simulink model "solar_mppt_hdl_ready"  (R2026a)
settings: Solver=FixedStepAuto  StopTime=1.0  FixedStep=1e-5
values from neighbouring files (symbols this model uses):
  irradiance_day = pchip(t_coarse, irradiance_coarse, t_sim)    [flc_init.m]
  t_sim = linspace(0, 1.0, 1001)    [flc_init.m]
undefined symbols (not defined in the file or in its folder): DiscIntNeverNeededParam
libraries: nesl_utility x5, fl_lib x4, ee_lib x2, sl_discontinuities x1
settings Model: Creator=user  LastModifiedBy=user
settings OptimizationCC: ConditionallyExecuteInputs=off
settings DebuggingCC: AlgebraicLoopMsg=error
settings HardwareCC: ProdHWDeviceType=ASIC/FPGA->ASIC/FPGA  TargetBitPerPointer=64.0  TargetBitPerSizeT=64.0  TargetBitPerPtrDiffT=64.0  TargetLongLongMode=on  TargetIntDivRoundTo=Zero  TargetEndianess=LittleEndian  TargetWordSize=64.0  TargetHWDeviceType=Custom Processor->MATLAB Host Computer  ProdEqTarget=off

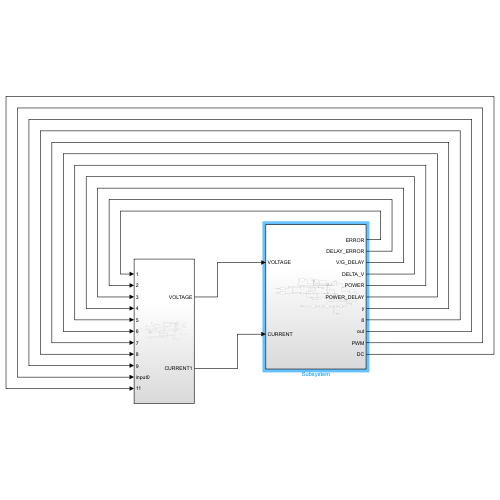
[thumbnail: Simulink's stored preview of the top-level diagram]
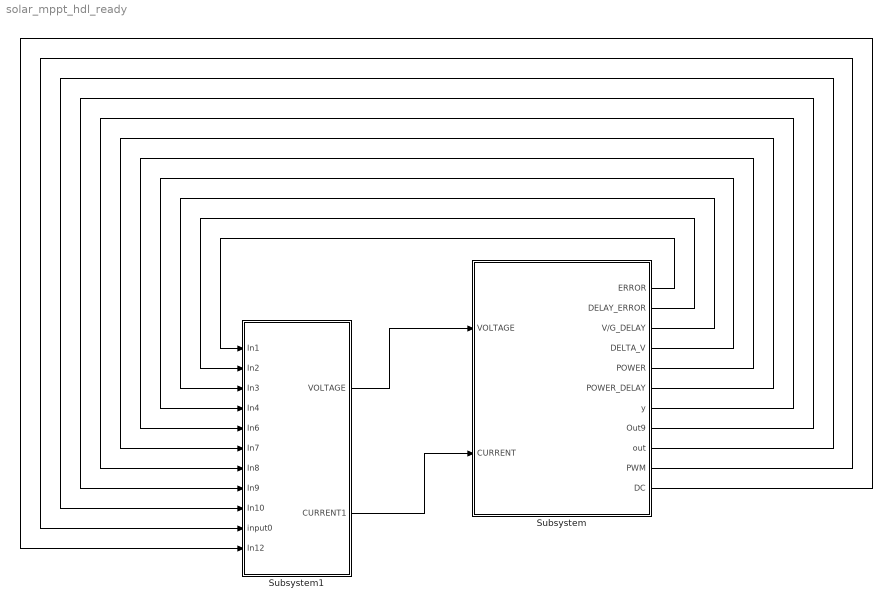
== system solar_mppt_hdl_ready ==
  Subsystem : Subsystem
  Subsystem1 : Subsystem
  wires:
  Subsystem/1(ERROR) -> Subsystem1/1(In1)
  Subsystem/2(DELAY_ERROR) -> Subsystem1/2(In2)
  Subsystem/3(V/G_DELAY) -> Subsystem1/3(In3)
  Subsystem/4(DELTA_V) -> Subsystem1/4(In4)
  Subsystem/5(POWER) -> Subsystem1/5(In6)
  Subsystem/6(POWER_DELAY) -> Subsystem1/6(In7)
  Subsystem/7(y) -> Subsystem1/7(In8)
  Subsystem/8(Out9) -> Subsystem1/8(In9)
  Subsystem/9(out) -> Subsystem1/9(In10)
  Subsystem/10(PWM) -> Subsystem1/10(input0)
  Subsystem/11(DC) -> Subsystem1/11(In12)
  Subsystem1/1(VOLTAGE) -> Subsystem/1(VOLTAGE)
  Subsystem1/2(CURRENT1) -> Subsystem/2(CURRENT)

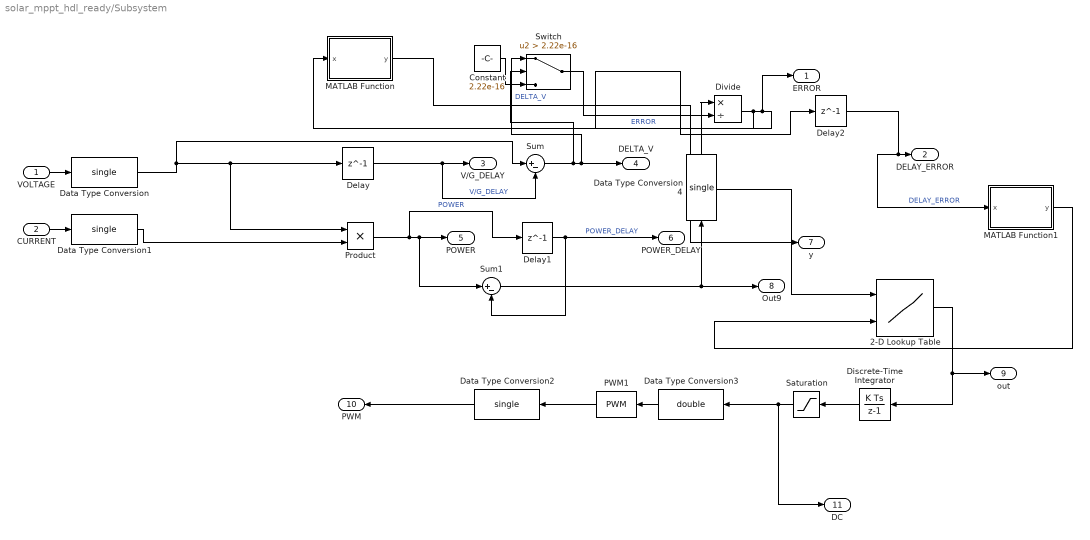
== system solar_mppt_hdl_ready/Subsystem ==
  VOLTAGE : Inport  SampleTime=1e-5
  CURRENT : Inport  Port=2  SampleTime=1e-5
  2-D Lookup Table : Lookup_n-D  BreakpointsForDimension1=[1:3]  BreakpointsForDimension2=[1:3]  InternalRulePriority=Speed  OutDataTypeStr=single  RndMeth=Simplest
      settings: InputPortMap=u0,u1
  Constant : Constant  Value=2.22e-16  OutDataTypeStr=single
  Data Type Conversion{,1..2,4} (4 alike) : DataTypeConversion  OutDataTypeStr=single  SaturateOnIntegerOverflow=off  RndMeth=Floor
  Data Type Conversion3 : DataTypeConversion  OutDataTypeStr=double  SaturateOnIntegerOverflow=off  RndMeth=Floor
  Delay : Delay  DelayLength=1  InitialCondition=0  InputProcessing=Columns as channels (frame based)
  Delay1 : Delay  DelayLength=1  InitialCondition=0  InputProcessing=Columns as channels (frame based)
  Delay2 : Delay  DelayLength=1  InitialCondition=0  InputProcessing=Columns as channels (frame based)
  Discrete-Time Integrator : DiscreteIntegrator  InitialCondition=0.4  SampleTime=-1  ICPrevOutput=DiscIntNeverNeededParam  ICPrevScaledInput=DiscIntNeverNeededParam
  Divide : Product  Inputs=*/
  MATLAB Function : MATLAB Function  TreatAsAtomicUnit=on
  MATLAB Function1 : MATLAB Function  TreatAsAtomicUnit=on
  PWM1 : sl_discontinuities/PWM  DisableCoverage=on  Period=1  InitialDelay=0  DisallowZeroDutyCycle=off  RunAtFixedTimeIntervals=on  SampleTime=1e-5
      settings: LibrarySourceBlock=simulink/Discontinuities/PWM
  Product : Product
  Saturation : Saturate  UpperLimit=0.9  LowerLimit=0.05  OutDataTypeStr=single
  Sum : Sum  Inputs=|+-
  Sum1 : Sum  Inputs=|+-
  Switch : Switch  Criteria=u2 > Threshold  Threshold=2.22e-16  SaturateOnIntegerOverflow=off  InputSameDT=off
  ERROR : Outport
  DELAY_ERROR : Outport  Port=2
  V/G_DELAY : Outport  Port=3
  DELTA_V : Outport  Port=4
  POWER : Outport  Port=5
  POWER_DELAY : Outport  Port=6
  y : Outport  Port=7
  Out9 : Outport  Port=8
  out : Outport  Port=9
  PWM : Outport  Port=10
  DC : Outport  Port=11
  wires:
  MATLAB Function/1(y) -> 2-D Lookup Table/1, y/1
  Discrete-Time Integrator/1 -> Saturation/1
  Saturation/1 -> Data Type Conversion3/1, DC/1
  MATLAB Function1/1(y) -> 2-D Lookup Table/2
  Sum/1 -> Switch/2, DELTA_V/1, Switch/1  "DELTA_V"
  Switch/1 -> Divide/2
  Delay1/1 -> POWER_DELAY/1, Sum1/2  "POWER_DELAY"
  Product/1 -> Delay1/1, POWER/1, Sum1/1  "POWER"
  Divide/1 -> MATLAB Function/1(x), ERROR/1, Delay2/1  "ERROR"
  Constant/1 -> Switch/3
  Sum1/1 -> Out9/1, Data Type Conversion4/1
  Delay/1 -> V/G_DELAY/1, Sum/2  "V/G_DELAY"
  PWM1/1 -> Data Type Conversion2/1
  2-D Lookup Table/1 -> out/1, Discrete-Time Integrator/1
  CURRENT/1 -> Data Type Conversion1/1
  Delay2/1 -> MATLAB Function1/1(x), DELAY_ERROR/1  "DELAY_ERROR"
  VOLTAGE/1 -> Data Type Conversion/1
  Data Type Conversion/1 -> Product/1, Delay/1, Sum/1
  Data Type Conversion1/1 -> Product/2
  Data Type Conversion3/1 -> PWM1/1
  Data Type Conversion2/1 -> PWM/1
  Data Type Conversion4/1 -> Divide/1

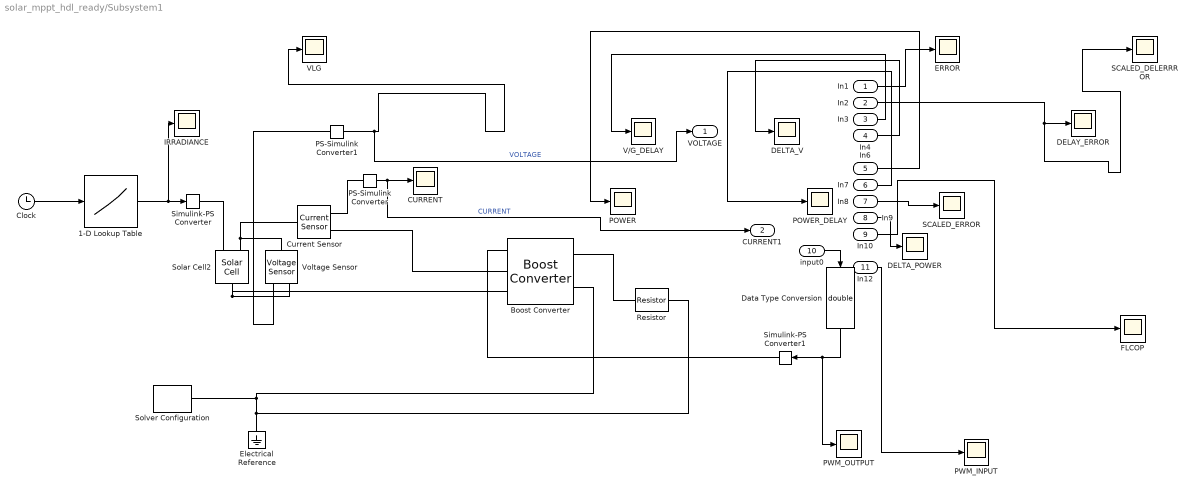
== system solar_mppt_hdl_ready/Subsystem1 ==
  In1 : Inport
  In2 : Inport  Port=2
  In3 : Inport  Port=3
  In4 : Inport  Port=4
  In6 : Inport  Port=5
  In7 : Inport  Port=6
  In8 : Inport  Port=7
  In9 : Inport  Port=8
  In10 : Inport  Port=9
  input0 : Inport  Port=10
  In12 : Inport  Port=11
  1-D Lookup Table : Lookup_n-D  NumberOfTableDimensions=1  BreakpointsForDimension1=t_sim  Table=irradiance_day  ExtrapMethod=Clip  InternalRulePriority=Speed  RndMeth=Simplest
  Boost Converter : ee_lib/Semiconductors & Converters/Converters/Boost Converter  port_option=ee.enum.controlport.ps  device_type=ee.enum.converters.switchingdevice.ideal  Vf=0.8 V  Ron=0.001 Ohm  Rds=0.001 Ohm  Goff=1e-5 1/Ohm  Vgt=1 V  Vgt_off=-1 V  Ih=1 A  Vth=6 V  K=0  diode_param=ee.enum.converters.protectiondiode.nodynamics  diode_Vf=0.8 V  diode_Ron=0.001 Ohm  diode_Goff=1e-5 1/Ohm  diode_C=50 nF  diode_iRM=-235 A  diode_iF=300 A  diode_idot=-50 A/us  diode_trr_param=ee.enum.converters.diodetrr.trr_factor  diode_trr_factor=3  diode_trr=15 us  diode_Qrr=1500 s*uA  Lf=1e-6 H  Rl=0 Ohm  Cf=1e-7 F  Rf=1e-6 Ohm  snubber_type=ee.enum.converters.snubber.exclude  Cs=1e-7 F  Rs=0.1 Ohm  iL_specify=off  iL_priority=High  iL=0 A  iL_nominal_specify=off  iL_nominal_value=1  iL_nominal_unit=A  vc_specify=off  vc_priority=High  vc=0 V  vc_nominal_specify=off  vc_nominal_value=1  vc_nominal_unit=V
  CURRENT : Scope
      settings: ActiveDisplayYMinimum=-0.41351020650465781  ActiveDisplayYMaximum=3.7215920776010369
  Clock : Clock
  Current Sensor : fl_lib/Electrical/Electrical Sensors/Current Sensor
  DELAY_ERROR : Scope
      settings: ActiveDisplayYMinimum=-0.932438052271241  ActiveDisplayYMaximum=7.5437756032088767  DataLoggingVariableName=ScopeData8
  DELTA_POWER : Scope
      settings: DataLoggingVariableName=ScopeData6
  DELTA_V : Scope
      settings: ActiveDisplayYMinimum=-1  ActiveDisplayYMaximum=1  DataLoggingVariableName=ScopeData3
  Data Type Conversion : DataTypeConversion  OutDataTypeStr=double  SaturateOnIntegerOverflow=off  RndMeth=Floor
  ERROR : Scope
      settings: ActiveDisplayYMinimum=-0.932438052271241  ActiveDisplayYMaximum=7.5437756032088767  DataLoggingVariableName=ScopeData7
  Electrical Reference : fl_lib/Electrical/Electrical Elements/Electrical Reference
  FLCOP : Scope
      settings: ActiveDisplayYMinimum=-1  ActiveDisplayYMaximum=1  DataLoggingVariableName=ScopeData9
  IRRADIANCE : Scope
      settings: ActiveDisplayYMinimum=-124.88690159999997  ActiveDisplayYMaximum=1124.9821144  DataLoggingVariableName=ScopeData16
  POWER : Scope
      settings: ActiveDisplayYMinimum=-1  ActiveDisplayYMaximum=1  DataLoggingVariableName=ScopeData4
  POWER_DELAY : Scope
      settings: Title=Output Power  ActiveDisplayYMinimum=-14.008631000583797  ActiveDisplayYMaximum=126.07767900525421  YLabel=Power Po(in watts)  DataLoggingVariableName=Po  DataLoggingSaveFormat=Array
  PS-Simulink Converter : nesl_utility/PS-Simulink Converter  PhysicalDomain=network_engine_domain  SubClassName=ps_output  LeftPortType=input  RightPortType=output  PseudoPeriodic=off  Frequencies=[]  VectorFormat=inherit  Unit=inherit  AffineConversion=off
  PS-Simulink Converter1 : nesl_utility/PS-Simulink Converter  PhysicalDomain=network_engine_domain  SubClassName=ps_output  LeftPortType=input  RightPortType=output  PseudoPeriodic=off  Frequencies=[]  VectorFormat=inherit  Unit=inherit  AffineConversion=off
  PWM_INPUT : Scope
      settings: ActiveDisplayYMinimum=-1  ActiveDisplayYMaximum=1  DataLoggingVariableName=ScopeData12
  PWM_OUTPUT : Scope
      settings: ActiveDisplayYMinimum=-1  ActiveDisplayYMaximum=1  DataLoggingVariableName=ScopeData11
  Resistor : fl_lib/Electrical/Electrical Elements/Resistor  R=10 Ohm  i_specify=off  i_priority=None  i=0 A  i_nominal_specify=off  i_nominal_value=1  i_nominal_unit=A  v_specify=off  v_priority=None  v=0 V  v_nominal_specify=off  v_nominal_value=1  v_nominal_unit=V
  SCALED_DELERRROR : Scope
      settings: ActiveDisplayYMinimum=-1  ActiveDisplayYMaximum=1  DataLoggingVariableName=ScopeData14
  SCALED_ERROR : Scope
      settings: ActiveDisplayYMinimum=-1  ActiveDisplayYMaximum=1  DataLoggingVariableName=ScopeData13
  Simulink-PS Converter : nesl_utility/Simulink-PS Converter  PhysicalDomain=network_engine_domain  SubClassName=ps_input  LeftPortType=input  RightPortType=output  PseudoPeriodic=off  Frequencies=[]  NoiseDistribution=none  NoiseParameters=[]  Unit=1  AffineConversion=off  FilteringAndDerivatives=provide  SimscapeFilterOrder=1  InputFilterTimeConstant=0.001  UdotUserProvided=0
  Simulink-PS Converter1 : nesl_utility/Simulink-PS Converter  PhysicalDomain=network_engine_domain  SubClassName=ps_input  LeftPortType=input  RightPortType=output  PseudoPeriodic=off  Frequencies=[]  NoiseDistribution=none  NoiseParameters=[]  Unit=1  AffineConversion=off  FilteringAndDerivatives=provide  SimscapeFilterOrder=1  InputFilterTimeConstant=0.001  UdotUserProvided=0
  Solar Cell2 : ee_lib/Sources/Solar Cell  prm=ee.enum.sources.solar_cell_prm.eightParameter  Isc=7.34 A  Voc=21.5 V  Is=1e-10 A  Is2=1e-10 A  Iph=7.34 A  Ir0=1000 W/m^2  ec=1.5  N2=2  Rs=0 Ohm  Rp=inf Ohm  N_series=36  N_parallel=1  TIPH1=0 1/K  EG=1.11 eV  TXIS1=3  TXIS2=3  TRS1=0  TRP1=0  Tmeas=25 degC  TFIXED=25 degC  thermal_mass=100 J/K  initial_temperature=25 degC
  Solver Configuration : nesl_utility/Solver Configuration  PhysicalDomain=network_engine_domain  SubClassName=solver  LeftPortType=input  RightPortType=generic  Tones=[]  Harmonics=[]  SimulateNoise=off  Profile=off  UseLocalSampling=off  EnableSwitchedLinearOptims=on  FrequencyDomain=off  UseCCode=off  RelTol=0.001  AbsTol=0.001  MinStep=1e-09  ToWorkspace=off  RevertToSquareIcSolve=off  NumHomotopyIterations=100  PhasorMode=off  PhasorModeNumHarmonics=1  ConsistencySolver=NEWTON_XTOL_AFTER_FTOL  CanonicalOrdering=CANONICAL  OptimizeIntermediates=OPTIMIZED  IndexReductionMethod=DerivativeReplacement  DoDC=off  ResidualTolerance=1e-09  ConsistencyTolSource=GLOBAL  ConsistencyAbsTol=0.001  ConsistencyRelTol=0.001  ConsistencyTolFactor=0.001  UseLocalSolver=off  LocalSolverChoice=NE_BACKWARD_EULER_ADVANCER  ResolveIndetEquations=on  FunctionEvalNumThread=1  LocalSolverSampleTime=0.001  DoFixedCost=off  MaxNonlinIter=3  MaxModeIter=2  ComputeImpulses=off  ImpulseIterations=2  LinearAlgebra=auto  LinearAlgebraNumThread=0  EquationFormulation=NE_TIME_EF  DelaysMemoryBudget=1024  AutomaticFiltering=on  FilteringTimeConstant=0.001  PartitionStorageMethod=AS_NEEDED  PartitionMemoryBudget=1024  PartitionMethod=ROBUST  MultibodyUseLocalSolver=off  MultibodyLocalSolverChoice=ODE1  MultibodyLocalSolverSampleTime=0.001
  V/G_DELAY : Scope
      settings: ActiveDisplayYMinimum=-4.2346688018048591  ActiveDisplayYMaximum=38.112019216243738  DataLoggingVariableName=ScopeData2
  VLG : Scope
      settings: Title=Output Voltage  ActiveDisplayYMinimum=-3.3265921205731632  ActiveDisplayYMaximum=38.011121807218  YLabel=Solar output voltage(V)  DataLoggingVariableName=ScopeData15
  Voltage Sensor : fl_lib/Electrical/Electrical Sensors/Voltage Sensor
  VOLTAGE : Outport
  CURRENT1 : Outport  Port=2
  wires:
  Clock/1 -> 1-D Lookup Table/1
  input0/1 -> Data Type Conversion/1
  PS-Simulink Converter/1 -> CURRENT1/1, CURRENT/1  "CURRENT"
  In6/1 -> POWER/1
  In3/1 -> V/G_DELAY/1
  In7/1 -> POWER_DELAY/1
  In2/1 -> SCALED_DELERRROR/1, DELAY_ERROR/1
  1-D Lookup Table/1 -> IRRADIANCE/1, Simulink-PS Converter/1
  In12/1 -> PWM_INPUT/1
  PS-Simulink Converter1/1 -> VOLTAGE/1, VLG/1  "VOLTAGE"
  In4/1 -> DELTA_V/1
  In1/1 -> ERROR/1
  In9/1 -> DELTA_POWER/1
  In10/1 -> FLCOP/1
  In8/1 -> SCALED_ERROR/1
  Data Type Conversion/1 -> PWM_OUTPUT/1, Simulink-PS Converter1/1
  connections:
  Boost Converter/LConn3 -- Solar Cell2/RConn1 -- Voltage Sensor/RConn2
  Boost Converter/RConn2 -- Electrical Reference/LConn1 -- Resistor/RConn1 -- Solver Configuration/RConn1
  Current Sensor/LConn1 -- Solar Cell2/LConn2 -- Voltage Sensor/LConn1
  Current Sensor/RConn2 -- Boost Converter/LConn2
  Simulink-PS Converter/RConn1 -- Solar Cell2/LConn1
  Simulink-PS Converter1/RConn1 -- Boost Converter/LConn1
  Current Sensor/RConn1 -- PS-Simulink Converter/LConn1
  Voltage Sensor/RConn1 -- PS-Simulink Converter1/LConn1
  Resistor/LConn1 -- Boost Converter/RConn1

== matlab function solar_mppt_hdl_ready/Subsystem/MATLAB Function ==
  data: x input; y output
function y = scaleValue(x)
    inMin = -0.5;
    inMax = 7.5;
    outMin = -1;
    outMax = 1;
    
    % Linear mapping
    scaled = outMin + ((x - inMin) / (inMax - inMin)) * (outMax - outMin);
    
    % Saturate the output between -1 and 1
    y = max(outMin, min(outMax, scaled));
end

== matlab function solar_mppt_hdl_ready/Subsystem/MATLAB Function1 ==
  data: x input; y output
function y = scaleValue(x)
    inMin = -0.5;
    inMax = 7.5;
    outMin = -1;
    outMax = 1;
    
    % Linear mapping
    scaled = outMin + ((x - inMin) / (inMax - inMin)) * (outMax - outMin);
    
    % Saturate the output between -1 and 1
    y = max(outMin, min(outMax, scaled));
end
